simulink model "system_model"  (R2025b)
settings: Solver=ode1  StartTime=0.0  StopTime=2  FixedStep=0.05  RelTol=1e-3
values from neighbouring files (symbols this model uses):
  p = params()    [Matlab_Test.m]    (also in detector.m = det.p; main.m; measurement_channel.m = mc.p)
settings Model: Creator=Dawid  LastModifiedBy=Dawid

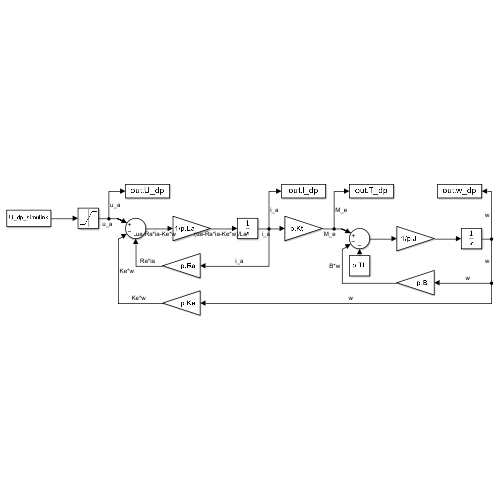
[thumbnail: Simulink's stored preview of the top-level diagram]
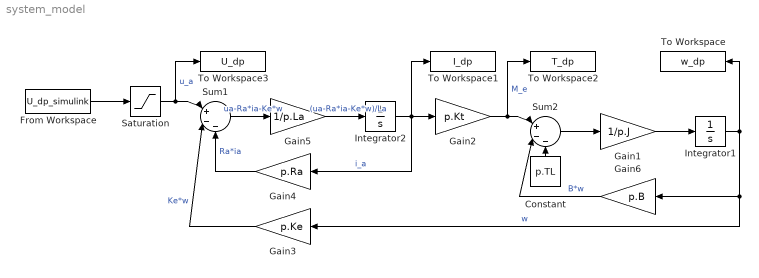
== system system_model ==
  Constant : Constant  Value=p.TL
  From Workspace : FromWorkspace  VariableName=U_dp_simulink  SampleTime=p.dt  Interpolate=off  OutputAfterFinalValue=Setting to zero
  Gain1 : Gain  Gain=1/p.J
  Gain2 : Gain  Gain=p.Kt
  Gain3 : Gain  Gain=p.Ke
  Gain4 : Gain  Gain=p.Ra
  Gain5 : Gain  Gain=1/p.La
  Gain6 : Gain  Gain=p.B
  Integrator1 : Integrator
  Integrator2 : Integrator
  Saturation : Saturate  UpperLimit=p.Umax  LowerLimit=p.Umin
  Sum1 : Sum  Inputs=|+--
  Sum2 : Sum  Inputs=|+--
  To Workspace : ToWorkspace  VariableName=w_dp  SaveFormat=Timeseries  SampleTime=-1
  To Workspace1 : ToWorkspace  VariableName=I_dp  SaveFormat=Timeseries  SampleTime=-1
  To Workspace2 : ToWorkspace  VariableName=T_dp  SaveFormat=Timeseries  SampleTime=-1
  To Workspace3 : ToWorkspace  VariableName=U_dp  SaveFormat=Timeseries  SampleTime=-1
  wires:
  From Workspace/1 -> Saturation/1
  Saturation/1 -> To Workspace3/1, Sum1/1  "u_a"
  Gain5/1 -> Integrator2/1  "(ua-Ra*ia-Ke*w)/La"
  Integrator2/1 -> To Workspace1/1, Gain4/1, Gain2/1  "i_a"
  Gain3/1 -> Sum1/2  "Ke*w"
  Gain2/1 -> To Workspace2/1, Sum2/1  "M_e"
  Sum2/1 -> Gain1/1
  Gain1/1 -> Integrator1/1
  Integrator1/1 -> Gain3/1, Gain6/1, To Workspace/1  "w"
  Gain4/1 -> Sum1/3  "Ra*ia"
  Sum1/1 -> Gain5/1  "ua-Ra*ia-Ke*w"
  Gain6/1 -> Sum2/2  "B*w"
  Constant/1 -> Sum2/3
